simulink model "DPWM_Modulation_Examples"  (R2024b)
settings: Solver=FixedStepDiscrete  StartTime=0.0  StopTime=0.1  FixedStep=5e-8  RelTol=1e-3
InitFcn:
  | Ts = 1/16000;
  | duty = 1;
settings Model: Creator=yqs  LastModifiedBy=yqs
settings DataIOCC: ReturnWorkspaceOutputs=off

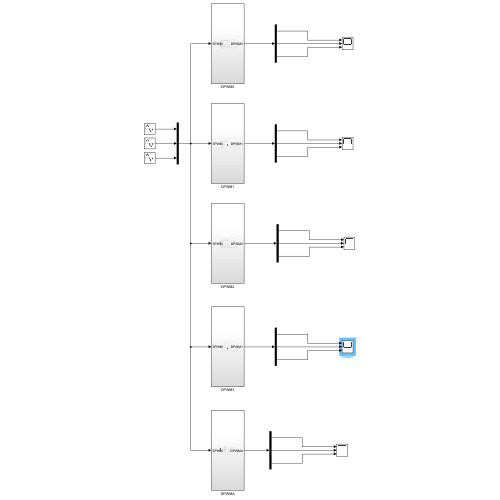
[thumbnail: Simulink's stored preview of the top-level diagram]
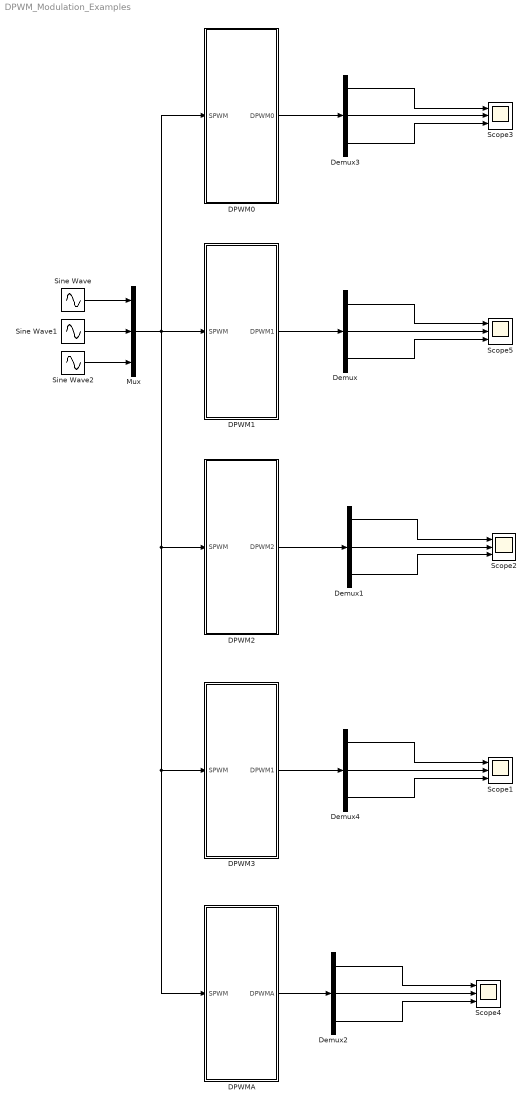
== system DPWM_Modulation_Examples ==
  DPWM0 : Subsystem
  DPWM1 : Subsystem
  DPWM2 : Subsystem
  DPWM3 : Subsystem
  DPWMA : Subsystem
  Demux{,1..4} (5 alike) : Demux  Outputs=3
  Mux : Mux  Inputs=3
  Scope{1..5} (5 alike) : Scope  NumInputPorts=3
  Sine Wave : Sin  Amplitude=duty  Frequency=100*pi  SampleTime=0
  Sine Wave1 : Sin  Amplitude=duty  Frequency=100*pi  Phase=2/3*pi  SampleTime=0
  Sine Wave2 : Sin  Amplitude=duty  Frequency=100*pi  Phase=-2/3*pi  SampleTime=0
  wires:
  Sine Wave1/1 -> Mux/2
  Sine Wave/1 -> Mux/1
  Sine Wave2/1 -> Mux/3
  DPWM1/1(DPWM1) -> Demux/1
  Demux/2 -> Scope5/2
  Demux/1 -> Scope5/1
  Demux/3 -> Scope5/3
  Demux2/3 -> Scope4/3
  Demux2/1 -> Scope4/1
  Demux2/2 -> Scope4/2
  DPWMA/1(DPWMA) -> Demux2/1
  DPWM2/1(DPWM2) -> Demux1/1
  Demux1/2 -> Scope2/2
  Demux1/1 -> Scope2/1
  Demux1/3 -> Scope2/3
  Demux3/3 -> Scope3/3
  Demux3/1 -> Scope3/1
  Demux3/2 -> Scope3/2
  DPWM0/1(DPWM0) -> Demux3/1
  Demux4/3 -> Scope1/3
  Demux4/1 -> Scope1/1
  Demux4/2 -> Scope1/2
  Mux/1 -> DPWM0/1(SPWM), DPWM3/1(SPWM), DPWMA/1(SPWM), DPWM2/1(SPWM), DPWM1/1(SPWM)
  DPWM3/1(DPWM1) -> Demux4/1

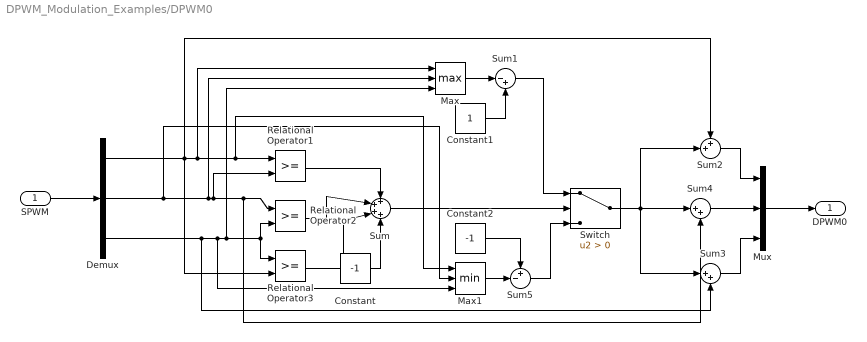
== system DPWM_Modulation_Examples/DPWM0 ==
  SPWM : Inport
  Constant : Constant  Value=-1
  Constant1 : Constant
  Constant2 : Constant  Value=-1
  Demux : Demux  Outputs=3
  Max : MinMax  Function=max  Inputs=3
  Max1 : MinMax  Inputs=3
  Mux : Mux  Inputs=3
  Relational Operator1 : RelationalOperator  OutDataTypeStr=boolean  RndMeth=Simplest  InputSameDT=off
  Relational Operator2 : RelationalOperator  OutDataTypeStr=boolean  RndMeth=Simplest  InputSameDT=off
  Relational Operator3 : RelationalOperator  OutDataTypeStr=boolean  RndMeth=Simplest  InputSameDT=off
  Sum : Sum  Inputs=++++
  Sum1 : Sum  Inputs=|-+
  Sum2 : Sum  Inputs=++|
  Sum3 : Sum  Inputs=|++
  Sum4 : Sum  Inputs=|++
  Sum5 : Sum  Inputs=+-|
  Switch : Switch  Criteria=u2 > Threshold  SaturateOnIntegerOverflow=off  InputSameDT=off
  DPWM0 : Outport
  wires:
  Sum5/1 -> Switch/3
  Constant2/1 -> Sum5/1
  Max1/1 -> Sum5/2
  Sum1/1 -> Switch/1
  Constant1/1 -> Sum1/2
  Max/1 -> Sum1/1
  Constant/1 -> Sum/4
  Sum/1 -> Switch/2
  Relational Operator3/1 -> Sum/3
  Relational Operator1/1 -> Sum/1
  Relational Operator2/1 -> Sum/2
  Sum3/1 -> Mux/3
  Sum2/1 -> Mux/1
  Mux/1 -> DPWM0/1
  Sum4/1 -> Mux/2
  Switch/1 -> Sum2/2, Sum3/1, Sum4/1
  SPWM/1 -> Demux/1
  Demux/1 -> Relational Operator3/2, Sum2/1, Relational Operator1/1, Max1/1, Max/1
  Demux/3 -> Sum3/2, Relational Operator2/2, Relational Operator3/1, Max/3, Max1/3
  Demux/2 -> Relational Operator1/2, Relational Operator2/1, Sum4/2, Max/2, Max1/2

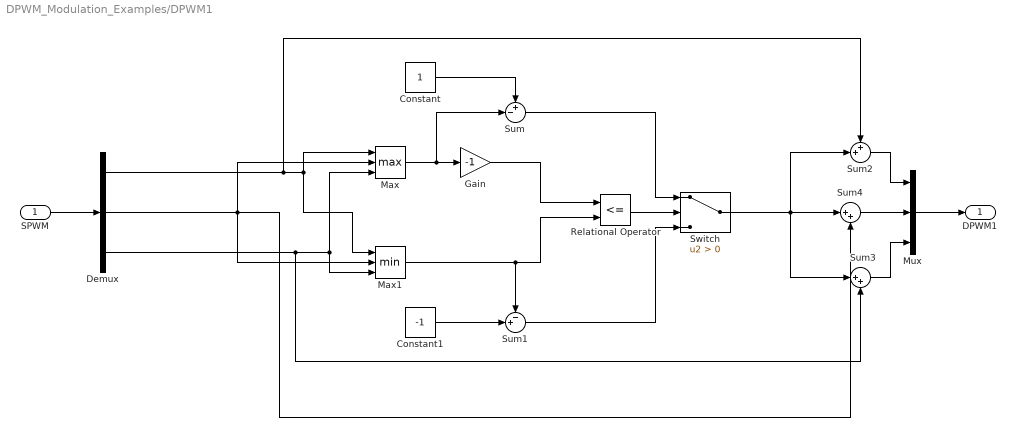
== system DPWM_Modulation_Examples/DPWM1 ==
  SPWM : Inport
  Constant : Constant
  Constant1 : Constant  Value=-1
  Demux : Demux  Outputs=3
  Gain : Gain  Gain=-1
  Max : MinMax  Function=max  Inputs=3
  Max1 : MinMax  Inputs=3
  Mux : Mux  Inputs=3
  Relational Operator : RelationalOperator  Operator=<=  OutDataTypeStr=boolean  RndMeth=Simplest  InputSameDT=off
  Sum : Sum  Inputs=+-|
  Sum1 : Sum  Inputs=-+|
  Sum2 : Sum  Inputs=++|
  Sum3 : Sum  Inputs=|++
  Sum4 : Sum  Inputs=|++
  Switch : Switch  Criteria=u2 > Threshold  SaturateOnIntegerOverflow=off  InputSameDT=off
  DPWM1 : Outport
  wires:
  Sum3/1 -> Mux/3
  Sum2/1 -> Mux/1
  Mux/1 -> DPWM1/1
  Sum4/1 -> Mux/2
  Switch/1 -> Sum2/2, Sum3/1, Sum4/1
  Sum1/1 -> Switch/3
  Constant1/1 -> Sum1/2
  Sum/1 -> Switch/1
  Constant/1 -> Sum/1
  Max/1 -> Gain/1, Sum/2
  Relational Operator/1 -> Switch/2
  SPWM/1 -> Demux/1
  Max1/1 -> Relational Operator/2, Sum1/1
  Gain/1 -> Relational Operator/1
  Demux/1 -> Max1/1, Max/1, Sum2/1
  Demux/3 -> Max1/3, Max/3, Sum3/2
  Demux/2 -> Max/2, Max1/2, Sum4/2

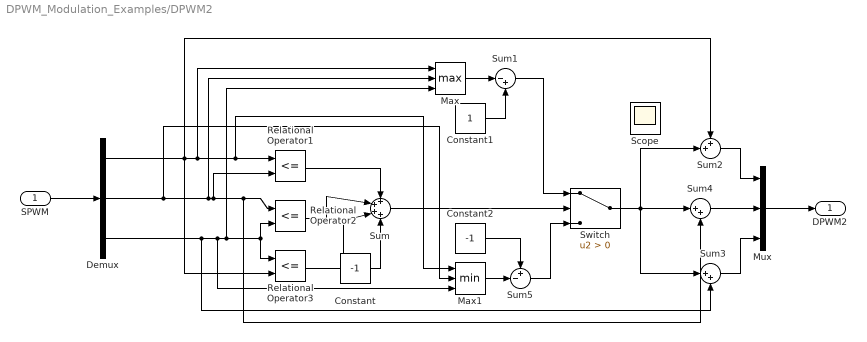
== system DPWM_Modulation_Examples/DPWM2 ==
  SPWM : Inport
  Constant : Constant  Value=-1
  Constant1 : Constant
  Constant2 : Constant  Value=-1
  Demux : Demux  Outputs=3
  Max : MinMax  Function=max  Inputs=3
  Max1 : MinMax  Inputs=3
  Mux : Mux  Inputs=3
  Relational Operator1 : RelationalOperator  Operator=<=  OutDataTypeStr=boolean  RndMeth=Simplest  InputSameDT=off
  Relational Operator2 : RelationalOperator  Operator=<=  OutDataTypeStr=boolean  RndMeth=Simplest  InputSameDT=off
  Relational Operator3 : RelationalOperator  Operator=<=  OutDataTypeStr=boolean  RndMeth=Simplest  InputSameDT=off
  Scope : Scope
  Sum : Sum  Inputs=++++
  Sum1 : Sum  Inputs=|-+
  Sum2 : Sum  Inputs=++|
  Sum3 : Sum  Inputs=|++
  Sum4 : Sum  Inputs=|++
  Sum5 : Sum  Inputs=+-|
  Switch : Switch  Criteria=u2 > Threshold  SaturateOnIntegerOverflow=off  InputSameDT=off
  DPWM2 : Outport
  wires:
  Demux/2 -> Max1/2, Max/2, Sum4/2, Relational Operator2/1, Relational Operator1/2
  Demux/3 -> Max1/3, Max/3, Relational Operator3/1, Relational Operator2/2, Sum3/2
  Demux/1 -> Max/1, Max1/1, Relational Operator1/1, Sum2/1, Relational Operator3/2
  SPWM/1 -> Demux/1
  Switch/1 -> Sum4/1, Sum3/1, Sum2/2
  Sum4/1 -> Mux/2
  Mux/1 -> DPWM2/1
  Sum2/1 -> Mux/1
  Sum3/1 -> Mux/3
  Relational Operator2/1 -> Sum/2
  Relational Operator1/1 -> Sum/1
  Relational Operator3/1 -> Sum/3
  Sum/1 -> Switch/2
  Constant/1 -> Sum/4
  ? -> Scope/1
  Max/1 -> Sum1/1
  Constant1/1 -> Sum1/2
  Sum1/1 -> Switch/1
  Max1/1 -> Sum5/2
  Constant2/1 -> Sum5/1
  Sum5/1 -> Switch/3

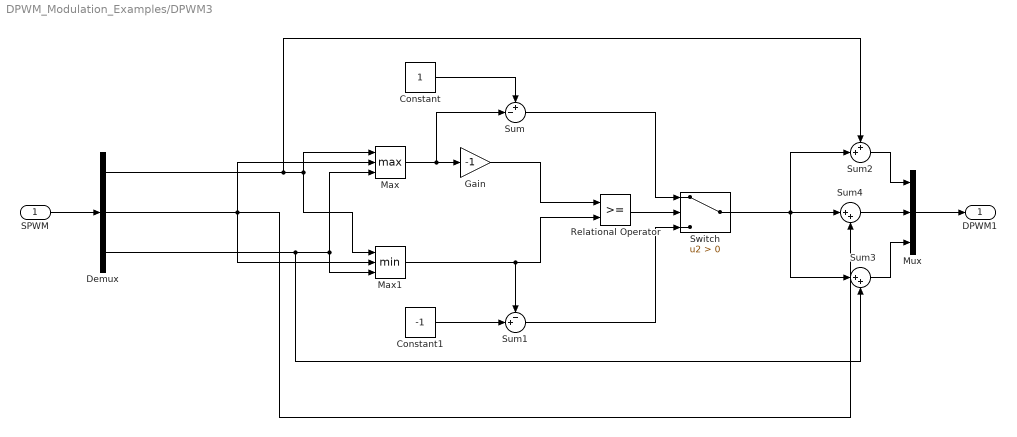
== system DPWM_Modulation_Examples/DPWM3 ==
  SPWM : Inport
  Constant : Constant
  Constant1 : Constant  Value=-1
  Demux : Demux  Outputs=3
  Gain : Gain  Gain=-1
  Max : MinMax  Function=max  Inputs=3
  Max1 : MinMax  Inputs=3
  Mux : Mux  Inputs=3
  Relational Operator : RelationalOperator  OutDataTypeStr=boolean  RndMeth=Simplest  InputSameDT=off
  Sum : Sum  Inputs=+-|
  Sum1 : Sum  Inputs=-+|
  Sum2 : Sum  Inputs=++|
  Sum3 : Sum  Inputs=|++
  Sum4 : Sum  Inputs=|++
  Switch : Switch  Criteria=u2 > Threshold  SaturateOnIntegerOverflow=off  InputSameDT=off
  DPWM1 : Outport
  wires:
  Sum3/1 -> Mux/3
  Sum2/1 -> Mux/1
  Mux/1 -> DPWM1/1
  Sum4/1 -> Mux/2
  Switch/1 -> Sum2/2, Sum3/1, Sum4/1
  Sum1/1 -> Switch/3
  Constant1/1 -> Sum1/2
  Sum/1 -> Switch/1
  Constant/1 -> Sum/1
  Max/1 -> Gain/1, Sum/2
  Relational Operator/1 -> Switch/2
  SPWM/1 -> Demux/1
  Max1/1 -> Relational Operator/2, Sum1/1
  Gain/1 -> Relational Operator/1
  Demux/1 -> Max1/1, Max/1, Sum2/1
  Demux/3 -> Max1/3, Max/3, Sum3/2
  Demux/2 -> Max/2, Max1/2, Sum4/2

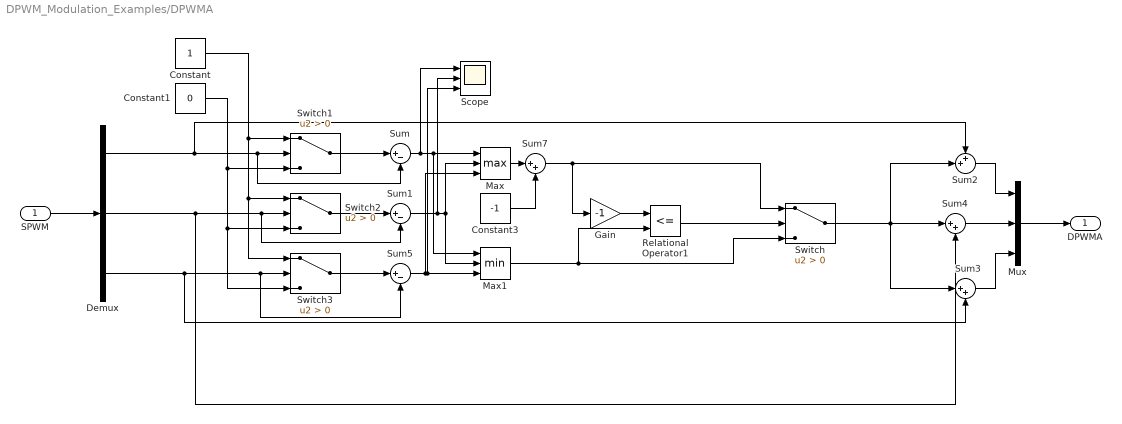
== system DPWM_Modulation_Examples/DPWMA ==
  SPWM : Inport
  Constant : Constant
  Constant1 : Constant  Value=0
  Constant3 : Constant  Value=-1
  Demux : Demux  Outputs=3
  Gain : Gain  Gain=-1
  Max : MinMax  Function=max  Inputs=3
  Max1 : MinMax  Inputs=3
  Mux : Mux  Inputs=3
  Relational Operator1 : RelationalOperator  Operator=<=  OutDataTypeStr=boolean  RndMeth=Simplest  InputSameDT=off
  Scope : Scope  NumInputPorts=3
  Sum : Sum  Inputs=|+-
  Sum1 : Sum  Inputs=|+-
  Sum2 : Sum  Inputs=++|
  Sum3 : Sum  Inputs=|++
  Sum4 : Sum  Inputs=|++
  Sum5 : Sum  Inputs=|+-
  Sum7 : Sum  Inputs=|++
  Switch{,1..3} (4 alike) : Switch  Criteria=u2 > Threshold  SaturateOnIntegerOverflow=off  InputSameDT=off
  DPWMA : Outport
  wires:
  Demux/2 -> Sum4/2, Switch2/2, Sum1/2
  SPWM/1 -> Demux/1
  Sum4/1 -> Mux/2
  Mux/1 -> DPWMA/1
  Sum2/1 -> Mux/1
  Sum3/1 -> Mux/3
  Demux/1 -> Sum/2, Switch1/2, Sum2/1
  Constant/1 -> Switch3/1, Switch2/1, Switch1/1
  Constant1/1 -> Switch3/3, Switch2/3, Switch1/3
  Demux/3 -> Sum5/2, Switch3/2, Sum3/2
  Switch1/1 -> Sum/1
  Switch2/1 -> Sum1/1
  Switch3/1 -> Sum5/1
  Sum/1 -> Scope/1, Max1/1, Max/1
  Sum1/1 -> Scope/2, Max/2, Max1/2
  Sum5/1 -> Max/3, Max1/3, Scope/3
  Max/1 -> Sum7/1
  Relational Operator1/1 -> Switch/2
  Switch/1 -> Sum3/1, Sum4/1, Sum2/2
  Max1/1 -> Relational Operator1/2, Switch/3
  Constant3/1 -> Sum7/2
  Sum7/1 -> Gain/1, Switch/1
  Gain/1 -> Relational Operator1/1
